simulink model "sm_car"  (R2025a)
settings: Solver=ode23t  StartTime=0.0  StopTime=400  MaxStep=0.4  RelTol=1e-3  AbsTol=1e-3  EnableMultiTasking=on
PreLoadFcn:
  | % Due to usability issue in Repeating Sequence block
  | warning('off','Simulink:Masking:Invalid');
  | 
  | % Eliminate unnecessary warnings in inactive variants
  | % Warnings generated only if you click through inactive variant
  | warning('off','MATLAB:nonExistentField');
  | warning('off','Simulink:Parameters:BlkParamUndefined');
PostLoadFcn:
  | set_param([bdroot '/Vehicle'],'popup_trailer','Off')
  | warning('off','sm:sli:setup:compile:LocalSolverNotSupported')
  | %sm_car_config_maneuver(bdroot,'WOT Braking');
  | sm_car_config_vehicle(bdroot,'false');
  | sm_car_config_logging(bdroot);
InitFcn:
  | sm_car_config_camera;
  | Vehicle = sm_car_vehcfg_checkConfig(Vehicle);
  | sm_car_check_tire_model(bdroot);
StartFcn:
  | tic;
StopFcn:
  | Elapsed_Sim_Time = toc;
  | % disp(['Elapsed Sim Time = ' num2str(Elapsed_Sim_Time)]);
undefined symbols (not defined in the file): Axle1D, AxleIn, Camera, Control, Driver, Free, Init, Maneuver, Pedal, RaceFix, RaceSpin, Scene, ShaftL1, ShaftL2, ShaftR1, ShaftR2, Soft, Stiff, Visual, X, xy_data_car_side, Y, Z
libraries: sm_lib x1546, nesl_utility x528, fl_lib x480, SimscapeFluids_lib x61, sdl_lib x49, simulink x29, ee_lib x7, simulink_extras x6, Linkage_Systems x4, Tire_1x2x x4, AntiRollBar_Systems x2, Linkage_Decoupled x2
(part 4 of 79)

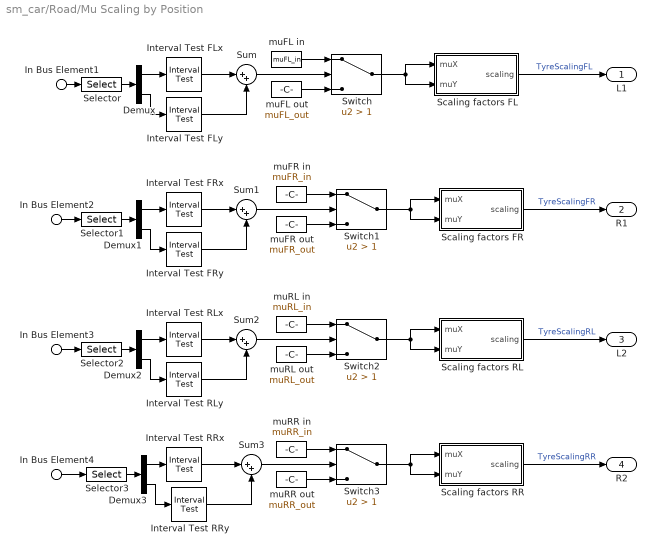
== system sm_car/Road/Mu Scaling by Position ==
  In Bus Element1 : Inport  PortName=Chassis  Element=WhlL1.xyz
  In Bus Element2 : Inport  PortName=Chassis  Element=WhlR1.xyz
  In Bus Element3 : Inport  PortName=Chassis  Element=WhlL2.xyz
  In Bus Element4 : Inport  PortName=Chassis  Element=WhlR2.xyz
  Demux{,1..3} (4 alike) : Demux  Outputs=2
  Interval Test FLx : simulink/Logic and Bit Operations/Interval Test  IntervalClosedRight=on  uplimit=intvX_FL_end  IntervalClosedLeft=on  lowlimit=intvX_FL_start  OutDataTypeStr=uint8
  Interval Test FLy : simulink/Logic and Bit Operations/Interval Test  IntervalClosedRight=on  uplimit=intvY_FL_end  IntervalClosedLeft=on  lowlimit=intvY_FL_start  OutDataTypeStr=uint8
  Interval Test FRx : simulink/Logic and Bit Operations/Interval Test  IntervalClosedRight=on  uplimit=intvX_FR_end  IntervalClosedLeft=on  lowlimit=intvX_FR_start  OutDataTypeStr=uint8
  Interval Test FRy : simulink/Logic and Bit Operations/Interval Test  IntervalClosedRight=on  uplimit=intvY_FR_end  IntervalClosedLeft=on  lowlimit=intvY_FR_start  OutDataTypeStr=uint8
  Interval Test RLx : simulink/Logic and Bit Operations/Interval Test  IntervalClosedRight=on  uplimit=intvX_RL_end  IntervalClosedLeft=on  lowlimit=intvX_RL_start  OutDataTypeStr=uint8
  Interval Test RLy : simulink/Logic and Bit Operations/Interval Test  IntervalClosedRight=on  uplimit=intvY_RL_end  IntervalClosedLeft=on  lowlimit=intvY_RL_start  OutDataTypeStr=uint8
  Interval Test RRx : simulink/Logic and Bit Operations/Interval Test  IntervalClosedRight=on  uplimit=intvX_RR_end  IntervalClosedLeft=on  lowlimit=intvX_RR_start  OutDataTypeStr=uint8
  Interval Test RRy : simulink/Logic and Bit Operations/Interval Test  IntervalClosedRight=on  uplimit=intvY_RR_end  IntervalClosedLeft=on  lowlimit=intvY_RR_start  OutDataTypeStr=uint8
  Scaling factors FL : Subsystem  mask{LKX=1, LKY=1, LKYC=1, LTR=1, LKZC=1}
      mask prompts: LKX "longitudinal slip stiffness"; LKY "cornering stiffness"; LKYC "camber stiffness"; LTR "pneumatic trail"; LKZC "camber torque stiffness"
  Scaling factors FR : Subsystem  mask{LKX=1, LKY=1, LKYC=1, LTR=1, LKZC=1}
      mask prompts: LKX "longitudinal slip stiffness"; LKY "cornering stiffness"; LKYC "camber stiffness"; LTR "pneumatic trail"; LKZC "camber torque stiffness"
  Scaling factors RL : Subsystem  mask{LKX=1, LKY=1, LKYC=1, LTR=1, LKZC=1}
      mask prompts: LKX "longitudinal slip stiffness"; LKY "cornering stiffness"; LKYC "camber stiffness"; LTR "pneumatic trail"; LKZC "camber torque stiffness"
  Scaling factors RR : Subsystem  mask{LKX=1, LKY=1, LKYC=1, LTR=1, LKZC=1}
      mask prompts: LKX "longitudinal slip stiffness"; LKY "cornering stiffness"; LKYC "camber stiffness"; LTR "pneumatic trail"; LKZC "camber torque stiffness"
  Selector{,1..3} (4 alike) : Selector  InputPortWidth=3  IndexOptions=Index vector (dialog)  Indices=[1 2]  OutputSizes=1
  Sum{,1..3} (4 alike) : Sum  Inputs=|++
  Switch : Switch  Criteria=u2 > Threshold  Threshold=1  ZeroCross=off  SaturateOnIntegerOverflow=off  InputSameDT=off
  Switch1 : Switch  Criteria=u2 > Threshold  Threshold=1  SaturateOnIntegerOverflow=off  InputSameDT=off
  Switch2 : Switch  Criteria=u2 > Threshold  Threshold=1  SaturateOnIntegerOverflow=off  InputSameDT=off
  Switch3 : Switch  Criteria=u2 > Threshold  Threshold=1  SaturateOnIntegerOverflow=off  InputSameDT=off
  muFL in : Constant  Value=muFL_in
  muFL out : Constant  Value=muFL_out
  muFR in : Constant  Value=muFR_in
  muFR out : Constant  Value=muFR_out
  muRL in : Constant  Value=muRL_in
  muRL out : Constant  Value=muRL_out
  muRR in : Constant  Value=muRR_in
  muRR out : Constant  Value=muRR_out
  L1 : Outport  VectorParamsAs1DForOutWhenUnconnected=off
  R1 : Outport  Port=2  VectorParamsAs1DForOutWhenUnconnected=off
  L2 : Outport  Port=3  VectorParamsAs1DForOutWhenUnconnected=off
  R2 : Outport  Port=4  VectorParamsAs1DForOutWhenUnconnected=off
  wires:
  Demux/1 -> Interval Test FLx/1
  Interval Test RRx/1 -> Sum3/1
  Demux3/2 -> Interval Test RRy/1
  Demux3/1 -> Interval Test RRx/1
  Sum3/1 -> Switch3/2
  Selector3/1 -> Demux3/1
  In Bus Element4/1 -> Selector3/1
  Interval Test RRy/1 -> Sum3/2
  Demux2/2 -> Interval Test RLy/1
  Selector2/1 -> Demux2/1
  Demux2/1 -> Interval Test RLx/1
  Interval Test RLy/1 -> Sum2/2
  Sum2/1 -> Switch2/2
  In Bus Element3/1 -> Selector2/1
  Interval Test RLx/1 -> Sum2/1
  Interval Test FRy/1 -> Sum1/2
  Selector1/1 -> Demux1/1
  Demux1/2 -> Interval Test FRy/1
  Sum1/1 -> Switch1/2
  Demux1/1 -> Interval Test FRx/1
  Interval Test FRx/1 -> Sum1/1
  Interval Test FLx/1 -> Sum/1
  Interval Test FLy/1 -> Sum/2
  Sum/1 -> Switch/2
  Demux/2 -> Interval Test FLy/1
  Selector/1 -> Demux/1
  muRR out/1 -> Switch3/3
  muRR in/1 -> Switch3/1
  Switch3/1 -> Scaling factors RR/2(muY), Scaling factors RR/1(muX)
  Scaling factors RR/1(scaling) -> R2/1  "TyreScalingRR"
  Scaling factors RL/1(scaling) -> L2/1  "TyreScalingRL"
  Switch2/1 -> Scaling factors RL/1(muX), Scaling factors RL/2(muY)
  muRL in/1 -> Switch2/1
  muRL out/1 -> Switch2/3
  muFR out/1 -> Switch1/3
  In Bus Element2/1 -> Selector1/1
  muFR in/1 -> Switch1/1
  Switch1/1 -> Scaling factors FR/2(muY), Scaling factors FR/1(muX)
  Scaling factors FR/1(scaling) -> R1/1  "TyreScalingFR"
  Scaling factors FL/1(scaling) -> L1/1  "TyreScalingFL"
  Switch/1 -> Scaling factors FL/1(muX), Scaling factors FL/2(muY)
  muFL out/1 -> Switch/3
  muFL in/1 -> Switch/1
  In Bus Element1/1 -> Selector/1

== system sm_car/Road/Road Surface Height ==
  Chassis : Inport
  None : Subsystem  VariantControl=None
  gz : Outport  VectorParamsAs1DForOutWhenUnconnected=off
  uvec : Outport  Port=2  VectorParamsAs1DForOutWhenUnconnected=off
  fcp : Outport  Port=3  VectorParamsAs1DForOutWhenUnconnected=off
  fco : Outport  Port=4  VectorParamsAs1DForOutWhenUnconnected=off
  fwc : Outport  Port=5  VectorParamsAs1DForOutWhenUnconnected=off

== system sm_car/Scopes/Subsystem ==
  In1 : Inport
  Bus Selector4 : BusSelector  OutputSignals=Chassis.Body.CG.vx,Chassis.Body.CG.vy,World.vx,World.vy,World.x,World.y
  Mux : Mux  Inputs=2
  Mux1 : Mux  Inputs=2
  Mux2 : Mux  Inputs=2
  Vel in xy plane : Fcn  Expr=sqrt(u(1)^2+u(2)^2)
  Vel in xy plane1 : Fcn  Expr=sqrt(u(1)^2+u(2)^2)
  Vel in xy plane2 : Fcn  Expr=sqrt(u(1)^2+u(2)^2)
  vBody : Outport  VectorParamsAs1DForOutWhenUnconnected=off
  vWorld : Outport  Port=2  VectorParamsAs1DForOutWhenUnconnected=off
  xWorld : Outport  Port=3  VectorParamsAs1DForOutWhenUnconnected=off
  wires:
  Bus Selector4/3 -> Mux1/1  "<vx>"
  Bus Selector4/4 -> Mux1/2  "<vy>"
  Bus Selector4/1 -> Mux/1  "<vx>"
  Vel in xy plane1/1 -> vWorld/1  "speed"
  In1/1 -> Bus Selector4/1
  Mux1/1 -> Vel in xy plane1/1
  Mux/1 -> Vel in xy plane/1
  Vel in xy plane/1 -> vBody/1  "speed"
  Bus Selector4/2 -> Mux/2  "<vy>"
  Mux2/1 -> Vel in xy plane2/1
  Bus Selector4/6 -> Mux2/2  "<y>"
  Bus Selector4/5 -> Mux2/1  "<x>"
  Vel in xy plane2/1 -> xWorld/1  "speed"

== system sm_car/Vehicle/Trailer ==
  "RdBus " : Inport
  "DrvBus " : Inport  Port=2
  "CtrlBus " : Inport  Port=3
  None : Subsystem  VariantControl=None
  " C" : PMIOPort  Side=Left
  " W" : PMIOPort  Port=2  Side=Left
  " Hitch" : PMIOPort  Port=3  Side=Right
  " VehBus" : Outport  VectorParamsAs1DForOutWhenUnconnected=off

== system sm_car/Vehicle/Vehicle ==
  In Bus Element2 : Inport  PortName=RdBus
  In Bus Element : Inport  Port=2  PortName=DrvBus
  In Bus Element3 : Inport  Port=2  PortName=DrvBus
  In Bus Element6 : Inport  Port=3  PortName=CtrlBus  Element=Brakes
  In Bus Element5 : Inport  Port=3  PortName=CtrlBus  Element=Chassis
  In Bus Element1 : Inport  Port=3  PortName=CtrlBus  Element=Power
  In Bus Element4 : Inport  Port=3  PortName=CtrlBus  Element=Driveline
  Body to World : Subsystem  Variant=on  VariantControlMode=label  VariantControl=Choice  LabelModeActiveChoice=Free  mask{popup_BodyToWorld=Free, SpecifyPosTarget=on}
      mask prompts: popup_BodyToWorld "Body To World Connection"; SpecifyPosTarget "Specify Position Target"
      mask init:
      | bh = gcb;
      | b2w = get_param(bh,'popup_BodyToWorld');
      | set_param(bh,'LabelModeActiveChoice',b2w)
      | if(strcmp(b2w,'Free'))
      |     set_param([bh '/Free'],'SpecifyPosTarget',get_param(bh,'SpecifyPosTarget'));
      | end
      mask TypeOptions popup_BodyToWorld: Free | Rigid
      mask Display: disp(' ')
  Brakes : Subsystem  Tag=PublishSubsystem  Variant=on  VariantControlMode=label  VariantControl=Variant1  LabelModeActiveChoice=PedalAbstract_DiscDisc  mask(Brake System){Brakes=Vehicle.Brakes, VariantLabel=Vehicle.Brakes.class.Value}
      mask prompts: Brakes "Brake Parameters"; VariantLabel "Variant Label"
      mask help: Select option and provide parameters for brakes. Option is chosen by string provided in Variant Label. The parameters for the selected option are contained in Brakes data structure.
      mask init:
      | curblk = gcb;
      | 
      | % Set variant for this block 
      | set_param(curblk,'LabelModeActiveChoice',VariantLabel);
      settings: AttributesFormatString=%<ActiveVariant>
  Chassis : Subsystem  Tag=PublishSubsystem  VariantControl=Chassis  mask(Chassis){Chassis=Vehicle.Chassis, Init=Init, mask_image_name=sm_car_vehicle_chassis_hamba_IMAGE.png, veh_index=veh_index}
      mask prompts: Chassis "Vehicle Parameters"; Init "Initial Values"; mask_image_name "Mask Image (string)"; veh_index "Vehicle Index (for tires)"
      mask help: Models vehicle chassis, with suspension, body, tires, springs, and dampers.
      mask Help: web('sm_car_doc_chassis.html')
      mask Display:
      | % Get image from BodyGeometry.class
      | % (active choice for Body Geometry subsystem)
      | temp_veh_bg_class = lower(get_param([gcb '/Body/Body Geometry'],'LabelModeActiveChoice'));
      | 
      | imagestr = (['sm_car_chassis_' temp_veh_bg_class '.png']);
      | if(~exist(imagestr))
      |     imagestr = ['sm_car_chassis_default.png'];
      | end
      | 
      | image(imagestr);
  Powertrain : Subsystem  mask(Powertrain, 2-Axle){Powertrain=Vehicle.Powertrain}
      mask prompts: Powertrain "Powertrain Parameters"
      mask help: Models power source and driveline for two-axle vehicles. The parameters for the selected options are contained in Powertrain data structure.
      mask Display: image('sm_car_vehicle_powertrain_IMAGE.png')
  Wheel Spin : Subsystem  Variant=on  VariantControlMode=label  VariantControl=Choice  LabelModeActiveChoice=Free  mask(Lock / Unlock Wheels){popup_wheel_spin=Free}
      mask prompts: popup_wheel_spin "Wheel Spin"
      mask help: For kinematics and compliance tests, the wheels need to be locked so they cannot spin. Leave unlocked for all other tests.
      mask init:
      | bh = gcb;
      | wspin = get_param(bh,'popup_wheel_spin');
      | set_param(bh,'LabelModeActiveChoice',wspin)
      settings: AttributesFormatString=%<popup_wheel_spin>
      mask TypeOptions popup_wheel_spin: Free | Lock
      mask Display: disp(' ')
  C : PMIOPort  Side=Left
  W : PMIOPort  Port=2  Side=Left
  HitchR : PMIOPort  Port=3  Side=Left
  HitchF : PMIOPort  Port=4  Side=Right
  Out Bus Elemet5 : Outport  VectorParamsAs1DForOutWhenUnconnected=off  PortName=VehBus  Element=Chassis
  Out Bus Element : Outport  VectorParamsAs1DForOutWhenUnconnected=off  PortName=VehBus  Element=Brakes
  Out Bus Element1 : Outport  VectorParamsAs1DForOutWhenUnconnected=off  PortName=VehBus  Element=Driveline
  Out Bus Element2 : Outport  VectorParamsAs1DForOutWhenUnconnected=off  PortName=VehBus  Element=World
  Out Bus Element3 : Outport  VectorParamsAs1DForOutWhenUnconnected=off  PortName=VehBus  Element=Power
  wires:
  In Bus Element5/1 -> Chassis/3(CtrlBus)
  Brakes/1(" OutB") -> Out Bus Element/1
  Chassis/1(VehBus) -> [VehB], Out Bus Elemet5/1
  In Bus Element2/1 -> Chassis/2(RdBus)
  In Bus Element/1 -> Chassis/1(DrvBus)
  In Bus Element6/1 -> Brakes/2("CtrlBus ")
  Body to World/1(World) -> Out Bus Element2/1
  In Bus Element3/1 -> Brakes/1("DrvBus ")
  In Bus Element4/1 -> Powertrain/1(CtrlD)
  In Bus Element1/1 -> Powertrain/2(CtrlP)
  Powertrain/1(OutD) -> Out Bus Element1/1
  Powertrain/2(OutP) -> Out Bus Element3/1
  [VehB] -> Powertrain/3(VehB)
  connections:
  Brakes/RConn2 -- Chassis/RConn6 -- Wheel Spin/RConn2 -- Powertrain/RConn4
  Chassis/RConn5 -- Powertrain/RConn3 -- Wheel Spin/RConn1 -- Brakes/RConn1
  HitchR/RConn1 -- Chassis/LConn1
  C/RConn1 -- Body to World/LConn1 -- Chassis/RConn1
  Body to World/RConn1 -- W/RConn1
  Brakes/LConn2 -- Chassis/LConn4 -- Wheel Spin/LConn2 -- Powertrain/LConn3
  Brakes/LConn1 -- Chassis/LConn3 -- Wheel Spin/LConn1 -- Powertrain/LConn2
  HitchF/RConn1 -- Chassis/RConn2
  Powertrain/LConn1 -- Chassis/LConn2
  Powertrain/RConn2 -- Chassis/RConn4
  Chassis/RConn3 -- Powertrain/RConn1

== system sm_car/Vehicle/Vehicle Constraint ==
  No Constraint : Subsystem  VariantControl=NoConstraint
  F : PMIOPort  Side=Right
  B : PMIOPort  Port=2  Side=Left

== system sm_car/Visualization/Dashboard ==
  VehBus : Inport
  DrvBus : Inport  Port=2
  Accelerator Pedal : LinearGaugeBlock  LabelPosition=Hide  ScaleMax=1  FontColor=[0.0, 0.0, 0.0]
  Brake Pedal : LinearGaugeBlock  ScaleMax=1  FontColor=[0.0, 0.0, 0.0]
  Bus Selector : BusSelector  OutputSignals=Chassis.Body.CG.vx
  Bus Selector2 : BusSelector  OutputSignals=aSteerWheel,rAccelPedal,rBrakePedal
  Gain : Gain  Gain=180/pi
  Gain1 : Gain  Gain=3.6
  Speed (kph) : CustomWebBlock  LabelPosition=Hide  ShowInitialText=on  Configuration="{\"components\":[{\"name\":\"CircularScaleComponent\",\"settings\":{\"bounds\":{\"max\":150,\"min\":0,\"tickInterval\":\"auto\"},\"direction\":\"cw\",\"flipLimits\":0,\"innerRadius\":0.46396628518311167,\"internalTickHeightScaleFactor\":1,\"labelColor\":[250,245,200],\"labelFont\":{\"font\":\"Arial\",\"fontSize\":12},\"labelRadius\":0.36,\"labelTransparency\":1,\"minorTickHeightScaleFactor\":0.2,\"needleImage\":{\"size\":[1890,567],\"src\":\"data:image\\/svg+xml;base64,PD94bWwgdmVyc2lvbj0iMS4wIiBlbmNvZGluZz0iVVRGLTgiIHN0YW5kYWxvbmU9Im5vIj8+CjxzdmcKICAgeG1sbnM6ZGM9Imh0dHA6Ly9wdXJsLm9yZy9kYy9lbGVtZW50cy8xLjEvIgogICB4bWxuczpjYz0iaHR0cDovL2NyZWF0aXZlY29tbW9ucy5vcmcvbnMjIgogICB4bWxuczpyZGY9Imh0dHA6Ly93d3cudzMub3JnLzE5OTkvMDIvMjItcmRmLXN5bnRheC1ucyMiCiAgIHhtbG5zOnN2Zz0iaHR0cDovL3d3dy53My5vcmcvMjAwMC9zdmciCiAgIHhtbG5zPSJodHRwOi8vd3d3LnczLm9yZy8yMDAwL3N2ZyIKICAgeG1sbnM6 ...(+4096 chars)\"},\"needleOffset\":[0.14,0],\"needleOrientation\":-45,\"needleRotation\":180,\"needleSize\":{\"height\":0.13,\"width\":0.41},\"outerRadius\":0.6228849068763098,\"position\":[0,0,1,1],\"scaleAngle\":299.999999999988,\"scaleAngleOffset\":119.46147497096791,\"scaleColors\":[],\"scaleColorsSize\":0.2,\"scalePosition\":[0,0,1,1],\"showLabels\":1,\"showMinorTicks\":1,\"showSpanLine\":1,\"showTicks\":1,\"tickColor\":[250,245,200],\"tickTransparency\":1,\"valueBarColor\":[23,89,176],\"valueBarPosition\":[0,0,1,1],\"valueBarSize\":0.2,\"valueBarTransparency\":1}},{\"name\":\"BackgroundImageComponent\",\"settings\":{\"image\":{\"size\":[500,500],\"src\":\"data:image\\/svg+xml;base64,PD94bWwgdmVyc2lvbj0iMS4wIiBlbmNvZGluZz0iVVRGLTgiIHN0YW5kYWxvbmU9Im5vIj8+CjwhLS0gR2VuZXJhdG9yOiBBZG9iZSBJbGx1c3RyYXRvciAxOS4yLjEsIFNWRyBFeHBvcnQgUGx1Zy1JbiAuIFNWRyBWZXJzaW9uOiA2LjAwIEJ1aWxkIDApICAtLT4KCjxzdmcKICAgeG1sbnM6ZGM9Imh0dHA6Ly9wdXJsLm9yZy9kYy9lbGVtZW50cy8xLjEvIgogICB4bWxuczpjYz0iaHR0cDovL2NyZWF0aXZlY29tbW9ucy5vcmcvbnMjIgogICB4bWxuczpyZGY9Imh0dHA6Ly93d3cudzMub3JnLzE5OTkvMDIvMjItcmRmLXN5bnRh ...(+9660 chars)\",\"srcOrientation\":\"horizontal\"},\"position\":[0,0,1,1],\"scaleMode\":\"0\"}},{\"name\":\"ForegroundImageComponent\",\"settings\":{\"image\":{\"size\":[0,0],\"src\":\"default\",\"srcOrientation\":[]},\"isForeground\":1,\"position\":[0,0,1,1],\"scaleMode\":\"0\"}}],\"settings\":{\"BindingType\":\"signal\",\"backgroundOffset\":0.14,\"backgroundOpacity\":1,\"fixedAspectRatio\":\"on\",\"orientation\":\"horizontal\",\"showBackgroundColor\":0},\"type\":\"CircularGauge\"}"
  Steering Wheel Angle : SemiCircularGaugeBlock  LabelPosition=Hide  ScaleMin=-80  ScaleMax=80  TickInterval=20  FontColor=[0.0, 0.0, 0.0]
  Terminator{,1..3} (4 alike) : Terminator
  wires:
  VehBus/1 -> Bus Selector/1
  DrvBus/1 -> Bus Selector2/1
  Bus Selector/1 -> Gain1/1  "<vx>"
  Gain/1 -> Terminator1/1  "aSteerWheel deg"
  Bus Selector2/3 -> Terminator3/1  "<rBrakePedal>"
  Bus Selector2/1 -> Gain/1  "<aSteerWheel>"
  Bus Selector2/2 -> Terminator2/1  "<rAccelPedal>"
  Gain1/1 -> Terminator/1  "Speed (kph)"

== system sm_car/Visualization/Data for Unreal ==
  VehBus : Inport
  DrvBus : Inport  Port=2
  Bus Selector : BusSelector  OutputSignals=aSteerWheel
  Bus Selector1 : BusSelector  OutputSignals=World.x,World.y,World.z  OutputAsBus=on
  Bus Selector2 : BusSelector  OutputSignals=World.aRoll,World.aPitch,World.aYaw  OutputAsBus=on
  Bus Selector5 : BusSelector  OutputSignals=Chassis.WhlL1.n,Chassis.WhlR1.n,Chassis.WhlL2.n,Chassis.WhlR2.n
  Bus Selector6 : BusSelector  OutputSignals=Chassis.WhlL1.aCamber,Chassis.WhlR1.aCamber,Chassis.WhlL2.aCamber,Chassis.WhlR2.aCamber
  Mux : Mux
  Mux1 : Mux
  xyz : Outport  VectorParamsAs1DForOutWhenUnconnected=off
  rpy : Outport  Port=2  VectorParamsAs1DForOutWhenUnconnected=off
  ws : Outport  Port=3  VectorParamsAs1DForOutWhenUnconnected=off
  aCamber : Outport  Port=4  VectorParamsAs1DForOutWhenUnconnected=off
  aSteerWheel : Outport  Port=5  VectorParamsAs1DForOutWhenUnconnected=off
  wires:
  Bus Selector/1 -> aSteerWheel/1  "<aSteerWheel>"
  Bus Selector6/4 -> Mux1/4  "<aCamber>"
  Bus Selector6/3 -> Mux1/3  "<aCamber>"
  Bus Selector6/2 -> Mux1/2  "<aCamber>"
  Mux/1 -> ws/1  "ws"
  Bus Selector2/1 -> rpy/1  "rpy"
  Bus Selector6/1 -> Mux1/1  "<aCamber>"
  Bus Selector5/1 -> Mux/1  "<n>"
  Bus Selector5/2 -> Mux/2  "<n>"
  Bus Selector5/4 -> Mux/4  "<n>"
  DrvBus/1 -> Bus Selector/1
  VehBus/1 -> Bus Selector1/1, Bus Selector2/1, Bus Selector5/1, Bus Selector6/1
  Mux1/1 -> aCamber/1  "aCamber"
  Bus Selector1/1 -> xyz/1  "xyz"
  Bus Selector5/3 -> Mux/3  "<n>"

== system sm_car/Visualization/Unreal ==
  "xyz " : Inport
  "rpy " : Inport  Port=2
  "ws " : Inport  Port=3
  "aCamber " : Inport  Port=4
  "aSteerWheel " : Inport  Port=5
  Animation Off : Subsystem  VariantControl=Off

== system sm_car/World/Mechanism Configuration ==
  Constant Gravity : Subsystem  VariantControl=ConstantGravity
  C : PMIOPort  Side=Right

== system sm_car/World/Scene ==
  CRG Hockenheim : Subsystem  VariantControl=CRG_Hockenheim  mask{geometry=Scene.CRG_Hockenheim.Geometry}
      mask prompts: geometry "Geometry (structure)"
  CRG Hockenheim F : Subsystem  VariantControl=CRG_Hockenheim_F  mask{geometry=Scene.CRG_Hockenheim_F.Geometry}
      mask prompts: geometry "Geometry (structure)"
  Plane Grid : Subsystem  VariantControl=Plane_Grid  mask{plane=Scene.Plane_Grid.Plane, grid=Scene.Plane_Grid.Grid}
      mask prompts: plane "Ground Plane (structure)"; grid "Grid (structure)"
  Skidpad : Subsystem  VariantControl=Skidpad  mask{circ_in=Scene.Skidpad.Circle_Inner, circ_out=Scene.Skidpad.Circle_Outer, plane=Scene.Skidpad.Plane}
      mask prompts: circ_in "Circle Inner (structure)"; circ_out "Circle Outer (structure)"; plane "Plane (structure)"
  W : PMIOPort  Side=Left
  Obs : Outport  VectorParamsAs1DForOutWhenUnconnected=off

== system sm_car/World/Visuals ==
  Off : Subsystem  VariantControl=Off
  W : PMIOPort  Side=Left

== system sm_car/Camera Frames/Dolly Camera/Off ==
  W : PMIOPort  Side=Left
  R : PMIOPort  Port=2  Side=Right
  connections:
  R/RConn1 -- W/RConn1

== system sm_car/Controller/Default/Brake Control ==
  "rBrakePedal " : Inport
  "VehBus " : Inport  Port=2
  Pedal : Subsystem  VariantControl=Pedal
  " Brakes" : Outport  VectorParamsAs1DForOutWhenUnconnected=off

== system sm_car/Controller/Default/Ctrl ==
  Bus Creator : BusCreator  Inputs=2
  Constant{,2..4} (4 alike) : Constant
  Mux : Mux  Inputs=2
  Mux1 : Mux  Inputs=2
  Ctrl : Outport
  wires:
  Constant3/1 -> Mux1/1  "RL"
  Constant4/1 -> Mux1/2  "RR"
  Constant2/1 -> Mux/2  "FR"
  Constant/1 -> Mux/1  "FL"
  Bus Creator/1 -> Ctrl/1  "Ctrl"
  Mux1/1 -> Bus Creator/2  "Axle2"
  Mux/1 -> Bus Creator/1  "Axle1"

== system sm_car/Controller/Default/Damper Control ==
  VehBus : Inport
  In Bus Element : Inport  Port=2  PortName=Ctrl  Element=Axle1
  In Bus Element1 : Inport  Port=2  PortName=Ctrl  Element=Axle2
  Bus Creator : BusCreator  Inputs=4
  Bus Selector : BusSelector  OutputSignals=Chassis.Damper.L1,Chassis.Damper.R1,Chassis.Damper.L2,Chassis.Damper.R2
  Damper Control A1 : Subsystem  Variant=on  VariantControlMode=label  VariantControl=Choice  LabelModeActiveChoice=None  mask(Damper Control, One Axle){popup_damper_control=None, ControlDamper=Control.Damper.Axle1}
      mask prompts: popup_damper_control "Damper Control"; ControlDamper "Control Parameters (structure)"
      mask help: Configurable damping control for left and right dampers.
      mask init:
      | bh = gcb;
      | set_param(bh,'LabelModeActiveChoice',get_param(bh,'popup_damper_control'));
      settings: AttributesFormatString=%<popup_damper_control>
      mask TypeOptions popup_damper_control: None | Coefficient | Force
      mask Display: disp(' ')
  Damper Control A2 : Subsystem  Variant=on  VariantControlMode=label  VariantControl=Choice  LabelModeActiveChoice=None  mask(Damper Control, One Axle){popup_damper_control=None, ControlDamper=Control.Damper.Axle2}
      mask prompts: popup_damper_control "Damper Control"; ControlDamper "Control Parameters (structure)"
      mask help: Configurable damping control for left and right dampers.
      mask init:
      | bh = gcb;
      | set_param(bh,'LabelModeActiveChoice',get_param(bh,'popup_damper_control'));
      settings: AttributesFormatString=%<popup_damper_control>
      mask TypeOptions popup_damper_control: None | Coefficient | Force
      mask Display: disp(' ')
  Damper : Outport
  wires:
  VehBus/1 -> Bus Selector/1
  Damper Control A1/1(L) -> Bus Creator/1  "L1"
  Bus Selector/1 -> Damper Control A1/1(mL)  "<L1>"
  Bus Selector/2 -> Damper Control A1/2(mR)  "<R1>"
  Bus Selector/3 -> Damper Control A2/1(mL)  "<L2>"
  Bus Selector/4 -> Damper Control A2/2(mR)  "<R2>"
  Bus Creator/1 -> Damper/1  "Damper"
  Damper Control A1/2(R) -> Bus Creator/2  "R1"
  Damper Control A2/1(L) -> Bus Creator/3  "L2"
  Damper Control A2/2(R) -> Bus Creator/4  "R2"
  In Bus Element/1 -> Damper Control A1/3(Inp)
  In Bus Element1/1 -> Damper Control A2/3(Inp)

== system sm_car/Controller/Default/Driveline Control ==
  Bus Creator : BusCreator  Inputs=1
  Constant : Constant  Value=0
  Driveline : Outport  VectorParamsAs1DForOutWhenUnconnected=off
  wires:
  Bus Creator/1 -> Driveline/1  "Driveline"
  Constant/1 -> Bus Creator/1  "placeholder"

== system sm_car/Controller/Default/Power Control ==
  note: For 4 Motor Powertrain only
  note: For 3&4 Motor Powertrain only
  note: Sign of target velocity is applied to torque request so that vehicle can drive forward or backward.
  rAccelPedal : Inport
  VehBus : Inport  Port=2
  vTgt : Inport  Port=3
  Bus Creator : BusCreator  Inputs=7
  Constant : Constant  Value=trq_ratio_front
  Constant1 : Constant  Value=0
  Constant2 : Constant  Value=1-trq_ratio_front
  Constant3 : Constant
  Constant4 : Constant  Value=-1
  Gain : Gain  Gain=trq_max
  Gain{1..4} (4 alike) : Gain  Gain=0.5
  Product : Product  Inputs=3
  Product1 : Product  Inputs=3
  Rate Limiter : RateLimiter  RisingSlewLimit=trq_rate_up  FallingSlewLimit=trq_rate_down  SampleTimeMode=inherited
  Switch : Switch  ZeroCross=off  SaturateOnIntegerOverflow=off  InputSameDT=off
  Terminator : Terminator
  Power : Outport  VectorParamsAs1DForOutWhenUnconnected=off
  wires:
  Bus Creator/1 -> Power/1  "Power"
  Product1/1 -> Gain2/1, Gain1/1, Bus Creator/4  "MMotorA2Demand"
  Gain/1 -> Rate Limiter/1
  Product/1 -> Bus Creator/1, Gain4/1, Gain3/1  "MMotorA1Demand"
  rAccelPedal/1 -> Gain/1
  VehBus/1 -> Terminator/1
  Constant1/1 -> Bus Creator/7  "MRegenBrakeLimit"
  Rate Limiter/1 -> Product1/1, Product/2
  Constant/1 -> Product/1
  Constant2/1 -> Product1/2
  Gain1/1 -> Bus Creator/5  "MMotorL2Demand"
  Gain2/1 -> Bus Creator/6  "MMotorR2Demand"
  Gain3/1 -> Bus Creator/2  "MMotorL1Demand"
  Gain4/1 -> Bus Creator/3  "MMotorR1Demand"
  vTgt/1 -> Switch/2
  Switch/1 -> Product/3, Product1/3  "Direction"
  Constant3/1 -> Switch/1
  Constant4/1 -> Switch/3

== system sm_car/Controller/Default/Spring Control ==
  VehBus : Inport
  In Bus Element : Inport  Port=2  PortName=Ctrl  Element=Axle1
  In Bus Element1 : Inport  Port=2  PortName=Ctrl  Element=Axle2
  Bus Creator : BusCreator  Inputs=4
  Bus Selector : BusSelector  OutputSignals=Chassis.Damper.L1,Chassis.Damper.R1,Chassis.Damper.L2,Chassis.Damper.R2
  Spring Control A1 : Subsystem  Variant=on  VariantControlMode=label  VariantControl=Choice  LabelModeActiveChoice=None  mask(Spring Control, One Axle){popup_spring_control=None, popup_gas_spring=Soft}
      mask prompts: popup_spring_control "Spring Control"; popup_gas_spring "Gas Spring"
      mask help: Configurable spring control for left and right sides.
      mask init:
      | bh = gcb;
      | set_param(bh,'LabelModeActiveChoice',get_param(bh,'popup_spring_control'));
      | set_param([bh '/Hydropneumatic'],'popup_gas_spring',get_param(bh,'popup_gas_spring'));
      mask TypeOptions popup_spring_control: None | Hydropneumatic
      mask Callback popup_spring_control:
      | bh = gcb;
      | maskObj = Simulink.Mask.get(bh); % Get the mask object of the current block
      | psg_h   = maskObj.getParameter('popup_gas_spring'); % Get the parameter to hide
      | 
      | % Check the value of ControlParam
      | controlParamValue = get_param(bh, 'popup_spring_control');
      | 
      | psg_h.Visible  = 'off';
      | 
      | if strcmp(controlParamValue, 'Hydropneumatic')
      |     psg_h.Visible  = 'on';
      | else
      |     psg_h.Visible  = 'off';
      | end
      mask TypeOptions popup_gas_spring: Stiff | Soft
      mask Display: disp(' ')
  Spring Control A2 : Subsystem  Variant=on  VariantControlMode=label  VariantControl=Choice  LabelModeActiveChoice=None  mask(Spring Control, One Axle){popup_spring_control=None, popup_gas_spring=Soft}
      mask prompts: popup_spring_control "Spring Control"; popup_gas_spring "Gas Spring"
      mask help: Configurable spring control for left and right sides.
      mask init:
      | bh = gcb;
      | set_param(bh,'LabelModeActiveChoice',get_param(bh,'popup_spring_control'));
      | set_param([bh '/Hydropneumatic'],'popup_gas_spring',get_param(bh,'popup_gas_spring'));
      mask TypeOptions popup_spring_control: None | Hydropneumatic
      mask Callback popup_spring_control:
      | bh = gcb;
      | maskObj = Simulink.Mask.get(bh); % Get the mask object of the current block
      | psg_h   = maskObj.getParameter('popup_gas_spring'); % Get the parameter to hide
      | 
      | % Check the value of ControlParam
      | controlParamValue = get_param(bh, 'popup_spring_control');
      | 
      | psg_h.Visible  = 'off';
      | 
      | if strcmp(controlParamValue, 'Hydropneumatic')
      |     psg_h.Visible  = 'on';
      | else
      |     psg_h.Visible  = 'off';
      | end
      mask TypeOptions popup_gas_spring: Stiff | Soft
      mask Display: disp(' ')
  Spring : Outport
  wires:
  VehBus/1 -> Bus Selector/1
  Spring Control A1/1(L) -> Bus Creator/1  "L1"
  Bus Selector/1 -> Spring Control A1/1(mL)  "<L1>"
  Bus Selector/2 -> Spring Control A1/2(mR)  "<R1>"
  Bus Selector/3 -> Spring Control A2/1(mL)  "<L2>"
  Bus Selector/4 -> Spring Control A2/2(mR)  "<R2>"
  Bus Creator/1 -> Spring/1  "Spring"
  Spring Control A1/2(R) -> Bus Creator/2  "R1"
  Spring Control A2/1(L) -> Bus Creator/3  "L2"
  Spring Control A2/2(R) -> Bus Creator/4  "R2"
  In Bus Element/1 -> Spring Control A1/3(Inp)
  In Bus Element1/1 -> Spring Control A2/3(Inp)

== system sm_car/Controller/Default/Susp ==
  aSteerWheel : Inport
  vx : Inport  Port=2
  Bus Creator1 : BusCreator  Inputs=1
  Bus Creator3 : BusCreator  Inputs=1
  Steer Axle 1 : Subsystem
  Steer Axle 2 : Subsystem
  SuspA1 : Outport  VectorParamsAs1DForOutWhenUnconnected=off
  SuspA2 : Outport  Port=2  VectorParamsAs1DForOutWhenUnconnected=off
  wires:
  Steer Axle 2/1(Steer) -> Bus Creator3/1
  Bus Creator1/1 -> SuspA1/1  "SuspA1"
  Steer Axle 1/1(Steer) -> Bus Creator1/1
  aSteerWheel/1 -> Steer Axle 1/1(aSteerWheel), Steer Axle 2/1(aSteerWheel)  "aSteerWheel"
  Bus Creator3/1 -> SuspA2/1  "SuspA2"
  vx/1 -> Steer Axle 2/2(vx), Steer Axle 1/2(vx)

== system sm_car/Controller/TrqVec 4Motor/Brake Control ==
  "rBrakePedal " : Inport
  "VehBus " : Inport  Port=2
  ABS : Subsystem  VariantControl=ABS  mask{abs_tire_radiusF=abs_tire_radiusF, abs_tire_radiusR=abs_tire_radiusR}
      mask prompts: abs_tire_radiusF "Tire Radius Front (m)"; abs_tire_radiusR "Tire Radius Rear (m)"
  Pedal : Subsystem  VariantControl=Pedal
  Pressure : Subsystem  VariantControl=Pressure
  " Brakes" : Outport  VectorParamsAs1DForOutWhenUnconnected=off

== system sm_car/Controller/TrqVec 4Motor/Ctrl ==
  Bus Creator : BusCreator  Inputs=2
  Constant{,2..4} (4 alike) : Constant
  Mux : Mux  Inputs=2
  Mux1 : Mux  Inputs=2
  Ctrl : Outport
  wires:
  Constant3/1 -> Mux1/1  "RL"
  Constant4/1 -> Mux1/2  "RR"
  Constant2/1 -> Mux/2  "FR"
  Constant/1 -> Mux/1  "FL"
  Bus Creator/1 -> Ctrl/1  "Ctrl"
  Mux1/1 -> Bus Creator/2  "Axle2"
  Mux/1 -> Bus Creator/1  "Axle1"

== system sm_car/Controller/TrqVec 4Motor/Damper Control ==
  VehBus : Inport
  In Bus Element : Inport  Port=2  PortName=Ctrl  Element=Axle1
  In Bus Element1 : Inport  Port=2  PortName=Ctrl  Element=Axle2
  Bus Creator : BusCreator  Inputs=4
  Bus Selector : BusSelector  OutputSignals=Chassis.Damper.L1,Chassis.Damper.R1,Chassis.Damper.L2,Chassis.Damper.R2
  Damper Control A1 : Subsystem  Variant=on  VariantControlMode=label  VariantControl=Choice  LabelModeActiveChoice=None  mask(Damper Control, One Axle){popup_damper_control=None, ControlDamper=Control.Damper.Axle1}
      mask prompts: popup_damper_control "Damper Control"; ControlDamper "Control Parameters (structure)"
      mask help: Configurable damping control for left and right dampers.
      mask init:
      | bh = gcb;
      | set_param(bh,'LabelModeActiveChoice',get_param(bh,'popup_damper_control'));
      settings: AttributesFormatString=%<popup_damper_control>
      mask TypeOptions popup_damper_control: None | Coefficient | Force
      mask Display: disp(' ')
  Damper Control A2 : Subsystem  Variant=on  VariantControlMode=label  VariantControl=Choice  LabelModeActiveChoice=None  mask(Damper Control, One Axle){popup_damper_control=None, ControlDamper=Control.Damper.Axle2}
      mask prompts: popup_damper_control "Damper Control"; ControlDamper "Control Parameters (structure)"
      mask help: Configurable damping control for left and right dampers.
      mask init:
      | bh = gcb;
      | set_param(bh,'LabelModeActiveChoice',get_param(bh,'popup_damper_control'));
      settings: AttributesFormatString=%<popup_damper_control>
      mask TypeOptions popup_damper_control: None | Coefficient | Force
      mask Display: disp(' ')
  Damper : Outport
  wires:
  VehBus/1 -> Bus Selector/1
  Damper Control A1/1(L) -> Bus Creator/1  "L1"
  Bus Selector/1 -> Damper Control A1/1(mL)  "<L1>"
  Bus Selector/2 -> Damper Control A1/2(mR)  "<R1>"
  Bus Selector/3 -> Damper Control A2/1(mL)  "<L2>"
  Bus Selector/4 -> Damper Control A2/2(mR)  "<R2>"
  Bus Creator/1 -> Damper/1  "Damper"
  Damper Control A1/2(R) -> Bus Creator/2  "R1"
  Damper Control A2/1(L) -> Bus Creator/3  "L2"
  Damper Control A2/2(R) -> Bus Creator/4  "R2"
  In Bus Element/1 -> Damper Control A1/3(Inp)
  In Bus Element1/1 -> Damper Control A2/3(Inp)

== system sm_car/Controller/TrqVec 4Motor/Driveline Control ==
  Bus Creator : BusCreator  Inputs=1
  Constant : Constant  Value=0
  Driveline : Outport  VectorParamsAs1DForOutWhenUnconnected=off
  wires:
  Bus Creator/1 -> Driveline/1  "Driveline"
  Constant/1 -> Bus Creator/1  "placeholder"
